simulink model "DCDC拓扑MATLAB仿真模型"  (R2024a)
settings: Solver=ode1  StartTime=0.0  StopTime=0.16  FixedStep=25e-9  MaxStep=5e-7  RelTol=1e-3
model workspace (MAT data in the model file):
  S.Coss = 1e-09
  S.Isat = 25
  S.L = 3.6e-06
  S.T_D1 = [0.71772271106 0.439813521831 0.439722845926 0.439659897498 0.439615651943 0.439584524223 0.439562966906 0.439548685103 0.439540182293 0.439536490281 0.43953700523 0.439541386891 ... (19375 elements, 25x25x31)]
  S.T_D2 = [0.717178349569 0.559937517176 0.55990263156 0.559878413607 0.55986139121 0.559849415613 0.559841122007 0.559835627482 0.559832356283 0.559830935922 0.559831134088 0.559832819881 ... (19375 elements, 25x25x31)]
  S.T_eta = [0 0 0 0 0 0 0 0 0 0 0 0 ... (19375 elements, 25x25x31)]
  S.T_fs = [30 40 75 100 125 150 200 200 200 250 250 275 ... (19375 elements, 25x25x31)]
  S.T_md = [1 1 1 1 1 1 1 1 1 1 1 1 ... (19375 elements, 25x25x31)]
  S.T_phi = [1.19741351569 0.500343703421 0.500483767979 0.500581010068 0.500649363857 0.500697454188 0.500730759931 0.500752825776 0.500765963418 0.500771668535 0.500770874014 0.500764105586 ... (19375 elements, 25x25x31)]
  S.T_pk = [1.33333333333 2.68942703114 2.73964726839 2.85027789077 2.90789704959 2.9409657645 2.48564279345 2.97524696494 3.12408185098 2.66060608601 2.77501889216 2.77086255768 ... (19375 elements, 25x25x31)]
  S.T_tr = [-1.33333333333 -2.68942703114 -2.73964726839 -2.85027789077 -2.90789704959 -2.9409657645 -2.48564279345 -2.97524696494 -3.12408185098 -2.66060608601 -2.77501889216 -2.77086255768 ... (19375 elements, 25x25x31)]
  S.bpIo = [0 0.5 1 1.5 2 2.5 3 3.5 4 4.5 5 5.5 6 6.5 7 7.5 8 8.5 9 9.5 10 10.5 11 11.5 12 12.5 13 13.5 14 14.5 15]
  S.bpVin = [24 25 26 27 28 29 30 31 32 33 34 35 36 37 38 39 40 41 42 43 44 45 46 47 48]
  S.bpVref = [24 25 26 27 28 29 30 31 32 33 34 35 36 37 38 39 40 41 42 43 44 45 46 47 48]
  S.cont1.method = 'Io-axis windowed re-solve'
  S.cont1.date = '2026-10-09'
  S.cont1.win = 'D2±0.06(扩0.15/全局), phi±5*w'
  S.cont1.skip = '等压族'
  S.dbn.policy = 'DBN4_policy'
  S.dbn.date = '2026-10-10'
  S.dbn.note = 'AI策略在线推理网格化'
  S.fsList = [30000 40000 50000 75000 100000 125000 150000 200000 250000 275000 300000]
  S.ilc.round = 1
  S.ilc.err_model = '0.054*|Vin-Vref|+0.13'
  S.ilc.lever = 'D2'
  S.ilc.date = '2026-10-09'
  S.ilc10.round = 10
  S.ilc10.basis = 'spot_def默认工况3.84A坑: 边界区D1-1q'
  S.ilc10.date = '2026-10-09'
  S.ilc11.round = 11
  S.ilc11.basis = 'spot_def阶跃平台5.74A: rows5.5/6.0 D1-1q'
  S.ilc11.date = '2026-10-09'
  S.ilc12.round = 12
  S.ilc12.basis = '真Io标定: 电阻切换负载下buck5.76A实测-3.84%'
  S.ilc12.date = '2026-10-10'
  S.ilc13.round = 13
  S.ilc13.basis = '断开后再平衡24.55(+2.28%)实测'
  S.ilc13.date = '2026-10-10'
  S.ilc2.round = 2
  S.ilc2.basis = '20点全矩阵实测'
  S.ilc2.date = '2026-10-09'
  S.ilc3.round = 3
  S.ilc3.basis = 'cal_sweep v2 17点(连续性重建表)'
  S.ilc3.date = '2026-10-09'
  S.ilc4.round = 4
  S.ilc4.basis = 'cal_sweep v3 17点残差'
  S.ilc4.date = '2026-10-09'
  S.ilc4.split = 'buck:D2x1.3; boost<2.3A:D2x1.0; boost>=2.3A:D1(死区换变量)'
  S.ilc5.round = 5
  S.ilc5.basis = 'cal_sweep v4 17点残差'
  S.ilc5.date = '2026-10-09'
  S.ilc5.detail = 'boost重载D1x2.0; buck边界4-5A加修D1; boost轻载量子踢q=25ns*fs'
  S.ilc6.round = 6
  S.ilc6.basis = 'cal_sweep v5 过冲点单量子反向'
  S.ilc6.date = '2026-10-09'
  S.ilc7.round = 7
  S.ilc7.basis = 'verify 20点终测残差'
  S.ilc7.date = '2026-10-09'
  S.ilc7.detail = 'boost row0.5 D2+2q; 对角列row0按verify误差修D2'
  S.ilc8.round = 8
  S.ilc8.basis = 'verify#2 boost轻载-5.0%过冲回调1q'
  S.ilc8.date = '2026-10-09'
  S.ilc9.round = '9c'
  S.ilc9.basis = '格点探测终选: D1净0q(+2.33%), 格距2.4V无±2%内格点'
  S.ilc9.date = '2026-10-09'
  S.td = 2e-07
  fsTab = [30 40 75 100 125 150 200 200 200 250 250 275 ... (625 elements, 25x25)]
undefined symbols (not defined in the file): DiscIntNeverNeededParam, L
libraries: spsVoltageMeasurementLib x7, spsSeriesRLCBranchLib x6, spsMosfetLib x4, spsCurrentMeasurementLib x3, spsMeanLib x2, eePowerMeasurement x2, slpidlib x1, spsDCVoltageSourceLib x1, sps_lib x1
settings Model: Creator=hp  LastModifiedBy=hp
settings DataIOCC: ReturnWorkspaceOutputs=off

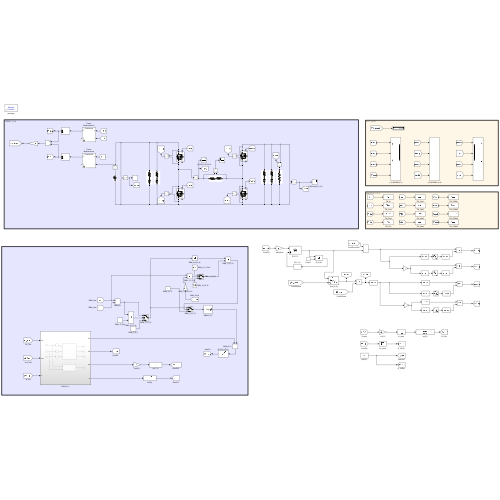
[thumbnail: Simulink's stored preview of the top-level diagram]
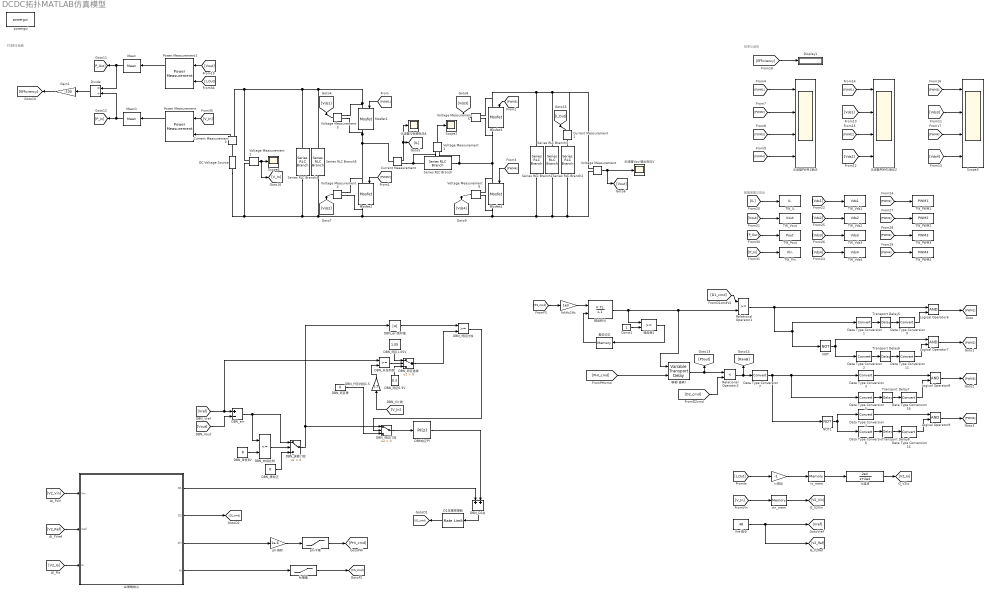
== system DCDC拓扑MATLAB仿真模型 ==
  note: FSBB主电路
  note: 效率与波形
  note: 数据收集与导出
  AI策略核心 : Subsystem
  Const1 : Constant
  Current Measurement : spsCurrentMeasurementLib/Current Measurement  PhasorSimulation=off  OutputType=Complex  PSBequivalent=0
  Current Measurement1 : spsCurrentMeasurementLib/Current Measurement  PhasorSimulation=off  OutputType=Complex  PSBequivalent=0
  Current Measurement2 : spsCurrentMeasurementLib/Current Measurement  PhasorSimulation=off  OutputType=Complex  PSBequivalent=0
  D1压摆率限制 : RateLimiter  RisingSlewLimit=50  FallingSlewLimit=-50  SampleTimeMode=inherited
  DBN_D1合 : Sum
  DBN_err : Sum  Inputs=+-
  DBN_err绝对值 : Abs  SaturateOnIntegerOverflow=off
  DBN_升压判别 : RelationalOperator  OutDataTypeStr=boolean  RndMeth=Simplest  InputSameDT=off
  DBN_升压判别1.5 : Gain  Gain=1.5
  DBN_带宽8V : Constant  Value=8
  DBN_死区0.3V : Constant  Value=0.3
  DBN_死区1.05V : Constant  Value=1.05
  DBN_死区比较 : RelationalOperator  OutDataTypeStr=boolean  RndMeth=Simplest  InputSameDT=off
  DBN_死区选择 : Switch  Criteria=u2 > Threshold  SaturateOnIntegerOverflow=off  InputSameDT=off
  DBN_死区门控 : Switch  Criteria=u2 > Threshold  SaturateOnIntegerOverflow=off  InputSameDT=off
  DBN_死区零 : Constant  Value=0
  DBN_误差门控 : Switch  Criteria=u2 > Threshold  SaturateOnIntegerOverflow=off  InputSameDT=off
  DBN_软启比较 : RelationalOperator  Operator=<=  OutDataTypeStr=boolean  RndMeth=Simplest  InputSameDT=off
  DBN_零校正 : Constant  Value=0
  DBN校正PI : slpidlib/PID Controller  Controller=PI  Form=Parallel  TimeDomain=Discrete-time  UseExternalTs=off  SampleTime=1e-5  IntegratorMethod=Forward Euler  FilterMethod=Forward Euler  ControllerParametersSource=internal  P=0.002  I=3  UseKiTs=off  D=0  UseExternalDerivativeSource=off  N=100  UseFilter=on  TunerSelectOption=Transfer Function Based (PID Tuner App)  InitialConditionSource=internal  InitialConditionForIntegrator=0  InitialConditionForFilter=0  DifferentiatorICPrevScaledInput=0  ExternalReset=none  TrackingMode=off  Kt=1  LimitOutput=on  SatLimitsSource=internal  UpperSaturationLimit=0.2  LowerSaturationLimit=-0.2  LinearizeAsGain=off  AntiWindupMode=none  Kb=1  LimitIntegrator=off  UpperIntegratorSaturationLimit=inf  LowerIntegratorSaturationLimit=-inf  POutMin=[]  POutMax=[]  IOutMin=[]  IOutMax=[]  DOutMin=[]  DOutMax=[]  NOutMin=[]  NOutMax=[]  SumOutMin=[]  SumOutMax=[]  SaturationOutMin=[]  SaturationOutMax=[]  PParamMin=[]  PParamMax=[]  IParamMin=[]  IParamMax=[]  DParamMin=[]  DParamMax=[]  NParamMin=[]  NParamMax=[]  KbParamMin=[]  KbParamMax=[]  KtParamMin=[]  KtParamMax=[]  KbOutMin=[]  KbOutMax=[]  KtOutMin=[]  KtOutMax=[]  IntegratorOutMin=[]  IntegratorOutMax=[]  FilterOutMin=[]  FilterOutMax=[]  SumI1OutMin=[]  SumI1OutMax=[]  SumI2OutMin=[]  SumI2OutMax=[]  SumI3OutMin=[]  SumI3OutMax=[]  SumI4OutMin=[]  SumI4OutMax=[]  SumDOutMin=[]  SumDOutMax=[]  DifferentiatorOutMin=[]  DifferentiatorOutMax=[]  FilterDiffOutCoefMin=[]  FilterDiffOutCoefMax=[]  ReciprocalOutMin=[]  ReciprocalOutMax=[]  SumDenOutMin=[]  SumDenOutMax=[]  SumNumOutMin=[]  SumNumOutMax=[]  DivideOutMin=[]  DivideOutMax=[]  UdiffTsProdOutMin=[]  UdiffTsProdOutMax=[]  NTsProdOutMin=[]  NTsProdOutMax=[]  UintegralTsProdOutMin=[]  UintegralTsProdOutMax=[]  UngainTsProdOutMin=[]  UngainTsProdOutMax=[]  ClampingZeroOutDataTypeStr=Inherit: Inherit via back propagation  ClampingZeroOutMin=[]  ClampingZeroOutMax=[]  FilterDenConstantOutDataTypeStr=Inherit: Inherit via back propagation  FilterDenConstantOutMin=[]  FilterDenConstantOutMax=[]  PCopyOutDataTypeStr=Inherit: Inherit via back propagation  PCopyOutMin=[]  PCopyOutMax=[]  NCopyOutDataTypeStr=Inherit: Inherit via back propagation  NCopyOutMin=[]  NCopyOutMax=[]  IntegratorContinuousStateAttributes=''  IntegratorStateMustResolveToSignalObject=off  IntegratorRTWStateStorageClass=Auto  FilterContinuousStateAttributes=''  FilterStateMustResolveToSignalObject=off  FilterRTWStateStorageClass=Auto  ParallelPVariant=InternalParameters  IdealPVariant=Disabled  IVariant=InternalParameters  DVariant=Disabled  IntegratorVariant=Discrete  SatVariant=Enabled  AWVariant=Passthrough  PCopyVariant=Disabled  TRVariant=Disabled  FdbkBlocksVariant=Forward  IdealPFdbkVariant=Disabled  SatFdbkVariant=Disabled  DerivativeFilterVariant=Disabled  NVariant=Disabled  NCopyVariant=Disabled_SignalSpec  FilterICVariant=Disabled  IntegratorICVariant=InternalICs  ExternalResetVariant=Disabled  TRSumVariant=Passthrough  SumFdbkVariant=Disabled  SumVariant=Sum_PI  TsampFilterVariant=InternalTs  TsampNgainVariant=Passthrough  TsampIntegralVariant=Disabled_SignalSpec  ExternalSaturationOutDataTypeStr=Inherit: Same as second input  DerivativeSourceVariant=Disabled
      settings: LibrarySourceBlock=simulink/Discrete/Discrete PID Controller
  DC Voltage Source : spsDCVoltageSourceLib/DC Voltage Source  Amplitude=48  Measurements=None
  Data Type Conversion{1..7,9,11,14,16} (11 alike) : DataTypeConversion  SaturateOnIntegerOverflow=off  RndMeth=Floor
  Display1 : Display
  Divide : Product  Inputs=*/
  Gain1 : Gain  Gain=-100
  Io滤波 : TransferFcn  Numerator=[2e4]  Denominator=[1 2e4]
  Logical Operator{6..9} (4 alike) : Logic  AllPortsSameDT=off  OutDataTypeStr=boolean
  Mean : spsMeanLib/Mean  Freq=50000  Vinit=0  Ts=0
  Mean1 : spsMeanLib/Mean  Freq=50000  Vinit=0  Ts=0
  Mosfet{1..4} (4 alike) : spsMosfetLib/Mosfet  Ron=4.4e-3  Lon=0  Rd=0.003  Vfd=1.5  IC=0  Rs=0.001  Cs=570e-12  Measurements=on
  NOT : Logic  Operator=NOT  IconShape=distinctive  AllPortsSameDT=off  OutDataTypeStr=boolean
  NOT1 : Logic  Operator=NOT  IconShape=distinctive  AllPortsSameDT=off  OutDataTypeStr=boolean
  Power Measurement : eePowerMeasurement/Power Measurement  LabelModeActiveChoice=Continuous  F=60  K=[0 1 2 3]  Ts=0
  Power Measurement1 : eePowerMeasurement/Power Measurement  LabelModeActiveChoice=Continuous  F=60  K=[0 1 2 3]  Ts=0
  Relational Operator1 : RelationalOperator  OutDataTypeStr=boolean  InputSameDT=off
  Relational Operator2 : RelationalOperator  Operator=<  OutDataTypeStr=boolean  InputSameDT=off
  Scope2 : Scope
  Scope3 : Scope  NumInputPorts=4
  Scope4 : Scope
  Series RLC Branch : spsSeriesRLCBranchLib/Series RLC Branch  LConnTagsString=__new0  RConnTagsString=__new0  BranchType=RL  Resistance=1.7e-3  Inductance=3.6e-6  SetiL0=off  InitialCurrent=0  Capacitance=1e-6  Setx0=off  InitialVoltage=0  Measurements=None
  Series RLC Branch1 : spsSeriesRLCBranchLib/Series RLC Branch  LConnTagsString=__new0  RConnTagsString=__new0  BranchType=RC  Resistance=2e-3  Inductance=1.5e-10  SetiL0=off  InitialCurrent=0  Capacitance=80e-6  Setx0=off  InitialVoltage=0  Measurements=Branch voltage and current
  Series RLC Branch2 : spsSeriesRLCBranchLib/Series RLC Branch  LConnTagsString=__new0  RConnTagsString=__new0  BranchType=R  Resistance=8  Inductance=L  SetiL0=off  InitialCurrent=0  Capacitance=1e-6  Setx0=off  InitialVoltage=0  Measurements=None
  Series RLC Branch3 : spsSeriesRLCBranchLib/Series RLC Branch  LConnTagsString=__new0  RConnTagsString=__new0  BranchType=RC  Resistance=0.09  Inductance=6e-9  SetiL0=off  InitialCurrent=0  Capacitance=3.667e-8  Setx0=off  InitialVoltage=0  Measurements=Branch voltage and current
  Series RLC Branch4 : spsSeriesRLCBranchLib/Series RLC Branch  LConnTagsString=__new0  RConnTagsString=__new0  BranchType=RC  Resistance=2e-3  Inductance=1.5e-10  SetiL0=off  InitialCurrent=0  Capacitance=50e-6  Setx0=off  InitialVoltage=0  Measurements=Branch voltage and current
  Series RLC Branch5 : spsSeriesRLCBranchLib/Series RLC Branch  LConnTagsString=__new0  RConnTagsString=__new0  BranchType=RC  Resistance=0.09  Inductance=6e-9  SetiL0=off  InitialCurrent=0  Capacitance=3.667e-8  Setx0=off  InitialVoltage=0  Measurements=Branch voltage and current
  TW_IL : ToWorkspace  VariableName=IL  SaveFormat=Timeseries  SampleTime=-1
  TW_PWM1 : ToWorkspace  VariableName=PWM1  SaveFormat=Timeseries  SampleTime=-1
  TW_PWM2 : ToWorkspace  VariableName=PWM2  SaveFormat=Timeseries  SampleTime=-1
  TW_PWM3 : ToWorkspace  VariableName=PWM3  SaveFormat=Timeseries  SampleTime=-1
  TW_PWM4 : ToWorkspace  VariableName=PWM4  SaveFormat=Timeseries  SampleTime=-1
  TW_Pin : ToWorkspace  VariableName=Pin  SaveFormat=Timeseries  SampleTime=-1
  TW_Pout : ToWorkspace  VariableName=Pout  SaveFormat=Timeseries  SampleTime=-1
  TW_Vds1 : ToWorkspace  VariableName=Vds1  SaveFormat=Timeseries  SampleTime=-1
  TW_Vds2 : ToWorkspace  VariableName=Vds2  SaveFormat=Timeseries  SampleTime=-1
  TW_Vds3 : ToWorkspace  VariableName=Vds3  SaveFormat=Timeseries  SampleTime=-1
  TW_Vds4 : ToWorkspace  VariableName=Vds4  SaveFormat=Timeseries  SampleTime=-1
  TW_Vout : ToWorkspace  VariableName=Vout  SaveFormat=Timeseries  SampleTime=-1
  Transport Delay{5..8} (4 alike) : TransportDelay  DelayTime=200e-9  BufferSize=500000
  Voltage Measurement{,1..6} (7 alike) : spsVoltageMeasurementLib/Voltage Measurement  PhasorSimulation=off  OutputType=Complex  PSBequivalent=0
  Vref指令 : Constant  Value=48
  fskHz2Hz : Gain  Gain=1e3
  fs限幅 : Saturate  UpperLimit=300  LowerLimit=30
  io_mem : Memory  InitialCondition=1
  io取反 : Gain  Gain=-1
  phi下限 : Saturate  UpperLimit=inf  LowerLimit=1e-7
  phi换秒 : Gain  Gain=1e-6
  powergui : sps_lib/powergui  Priority=1  SimulationMode=Discrete  SampleTime=25e-9  frequency=60  Iterations=50  frequencyindice=0  Pbase=100e6  ErrMax=1e-4  UnitsV=kV  UnitsW=MW  buscounter=0  FunctionMessages=off  echomessages=off  EnableUseOfTLC=off  CurrentSourceSwitches=off  DisableSnubberDevices=off  DisableRonSwitches=off  DisableVfSwitches=off  DisplayEquations=off  AutomaticDiscreteSolvers=off  SolverType=Tustin/Backward Euler (TBE)  Interpol=off  ExternalGateDelay=off  methode=off  Ts=100  x0status=blocks  SPID=on  SwTol=0  HookPort=off  NonlinearTolerance=1e-4  nMaxIteration=100  ContinueOnMaxIteration=off  RestoreLinks=warning  ResistiveCurrentMeasurement=off  Frange=[0:2:500]  Ylog=off  Xlog=on  ShowGrid=off  save=off  variable=ZData  structure=0  ZoomFFT=off  StartTime=0.0  cycles=1  DisplayStyle=1  fundamental=60  FreqAxis=off  MaxFrequency=1000  frequencyindicesteady=1  RmsSteady=1  display=off
  vin_mem : Memory  InitialCondition=48
  复位记忆 : Memory
  示波器IL电感电流A : Scope
  示波器PWM1驱动 : Scope  NumInputPorts=4
  示波器PWM1驱动2 : Scope  NumInputPorts=4
  示波器Vout输出电压V : Scope
  移相(查表) : VariableTransportDelay  VariableDelayType=Variable transport delay  MaximumDelay=1e-5
  锯齿满1 : RelationalOperator  OutDataTypeStr=boolean  RndMeth=Simplest  InputSameDT=off
  锯齿积分 : DiscreteIntegrator  gainval=1  ExternalReset=rising  SampleTime=25e-9  ICPrevOutput=DiscIntNeverNeededParam  ICPrevScaledInput=DiscIntNeverNeededParam
  wires:
  Voltage Measurement/1 -> [Vout], 示波器Vout输出电压V/1
  Current Measurement/1 -> [IL], 示波器IL电感电流A/1
  Voltage Measurement1/1 -> Scope2/1
  Voltage Measurement2/1 -> [V_In], Scope4/1
  [PWM2] -> Mosfet2/1
  [PWM4] -> Mosfet4/1
  [PWM3] -> Mosfet3/1
  Transport Delay5/1 -> Data Type Conversion9/1
  Data Type Conversion9/1 -> Logical Operator6/2
  Logical Operator6/1 -> [PWM1]
  Transport Delay6/1 -> Data Type Conversion11/1
  Data Type Conversion11/1 -> Logical Operator7/2
  Logical Operator7/1 -> [PWM2]
  Logical Operator9/1 -> [PWM4]
  Logical Operator8/1 -> [PWM3]
  Transport Delay7/1 -> Data Type Conversion16/1
  Transport Delay8/1 -> Data Type Conversion14/1
  Data Type Conversion16/1 -> Logical Operator8/2
  Data Type Conversion14/1 -> Logical Operator9/2
  NOT1/1 -> Data Type Conversion6/1, Data Type Conversion4/1
  Relational Operator1/1 -> Logical Operator6/1, Data Type Conversion1/1, NOT/1
  NOT/1 -> Logical Operator7/1, Data Type Conversion2/1
  Data Type Conversion3/1 -> Logical Operator8/1
  Data Type Conversion4/1 -> Logical Operator9/1
  Data Type Conversion1/1 -> Transport Delay5/1
  Data Type Conversion2/1 -> Transport Delay6/1
  Data Type Conversion5/1 -> Transport Delay7/1
  Data Type Conversion6/1 -> Transport Delay8/1
  [PWM1] -> Mosfet1/1
  Current Measurement2/1 -> Power Measurement/2
  Power Measurement1/1 -> Mean/1
  Power Measurement/1 -> Mean1/1
  Mean1/1 -> [P_In], Divide/2
  Mean/1 -> [P_Out], Divide/1
  Divide/1 -> Gain1/1
  [PWM1] -> 示波器PWM1驱动/1
  [PWM2] -> 示波器PWM1驱动/2
  [PWM3] -> 示波器PWM1驱动/3
  [PWM4] -> 示波器PWM1驱动/4
  Voltage Measurement3/1 -> [Vds1]
  Voltage Measurement4/1 -> [Vds2]
  Voltage Measurement5/1 -> [Vds3]
  [PWM1] -> 示波器PWM1驱动2/1
  [Vds1] -> 示波器PWM1驱动2/2
  [PWM2] -> 示波器PWM1驱动2/3
  [Vds2] -> 示波器PWM1驱动2/4
  [Vds4] -> Scope3/4
  [PWM4] -> Scope3/3
  [Vds3] -> Scope3/2
  [PWM3] -> Scope3/1
  Gain1/1 -> [Efficiency]
  [Efficiency] -> Display1/1
  移相(查表)/1 -> Relational Operator2/1, [PSout]
  Relational Operator2/1 -> Data Type Conversion7/1, [RawB]
  Data Type Conversion7/1 -> Data Type Conversion5/1, Data Type Conversion3/1, NOT1/1
  [D2_cmd] -> Relational Operator2/2
  [PHI_cmd] -> 移相(查表)/2
  [Vout] -> Power Measurement1/1
  [IL] -> TW_IL/1
  [Vout] -> TW_Vout/1
  [Vds1] -> TW_Vds1/1
  [Vds2] -> TW_Vds2/1
  [Vds3] -> TW_Vds3/1
  [Vds4] -> TW_Vds4/1
  [PWM1] -> TW_PWM1/1
  [PWM2] -> TW_PWM2/1
  [PWM3] -> TW_PWM3/1
  [PWM4] -> TW_PWM4/1
  [P_In] -> TW_Pin/1
  [P_Out] -> TW_Pout/1
  Current Measurement1/1 -> [I_Out]
  [I_Out] -> Power Measurement1/2
  [V_In] -> Power Measurement/1
  Voltage Measurement6/1 -> [Vds4]
  [D1_cmd] -> Relational Operator1/1
  [I_Out] -> io取反/1
  io_mem/1 -> Io滤波/1
  Io滤波/1 -> [V2_Io]
  [V_In] -> vin_mem/1
  vin_mem/1 -> [V2_Vin]
  Vref指令/1 -> [Vref], [V2_Ref]
  fs限幅/1 -> [FS_cmd]
  phi换秒/1 -> phi下限/1
  phi下限/1 -> [PHI_cmd]
  [FS_cmd] -> fskHz2Hz/1
  fskHz2Hz/1 -> 锯齿积分/1
  锯齿积分/1 -> 锯齿满1/1, 移相(查表)/1, Relational Operator1/2
  Const1/1 -> 锯齿满1/2
  锯齿满1/1 -> 复位记忆/1
  复位记忆/1 -> 锯齿积分/2
  io取反/1 -> io_mem/1
  [Vref] -> DBN_升压判别/1, DBN_err/1
  [Vout] -> DBN_err/2
  AI策略核心/1(D1) -> DBN_D1合/1
  AI策略核心/2(D2) -> [D2_cmd]
  AI策略核心/3(phi) -> phi换秒/1
  AI策略核心/4(fs) -> fs限幅/1
  [V2_Vin] -> AI策略核心/1(Vin)
  [V2_Ref] -> AI策略核心/2(Vref)
  [V2_Io] -> AI策略核心/3(Io)
  DBN_软启比较/1 -> DBN_误差门控/2
  DBN_零校正/1 -> DBN_误差门控/3
  DBN_D1合/1 -> D1压摆率限制/1
  D1压摆率限制/1 -> [D1_cmd]
  DBN_err/1 -> DBN_误差门控/1, DBN_软启比较/1
  DBN_带宽8V/1 -> DBN_软启比较/2
  DBN校正PI/1 -> DBN_D1合/2
  DBN_误差门控/1 -> DBN_err绝对值/1, DBN_死区门控/1
  DBN_死区零/1 -> DBN_死区门控/3
  DBN_死区门控/1 -> DBN校正PI/1
  [V_In] -> DBN_升压判别1.5/1
  DBN_升压判别1.5/1 -> DBN_升压判别/2
  DBN_死区1.05V/1 -> DBN_死区选择/1
  DBN_死区0.3V/1 -> DBN_死区选择/3
  DBN_升压判别/1 -> DBN_死区选择/2
  DBN_死区选择/1 -> DBN_死区比较/2
  DBN_err绝对值/1 -> DBN_死区比较/1
  DBN_死区比较/1 -> DBN_死区门控/2
  connections:
  Series RLC Branch2/RConn1 -- Voltage Measurement/LConn2 -- Series RLC Branch3/RConn1 -- Voltage Measurement6/LConn2 -- Mosfet4/RConn1 -- Voltage Measurement4/LConn2 -- Mosfet2/RConn1 -- Series RLC Branch5/RConn1 -- Series RLC Branch4/RConn1 -- Voltage Measurement2/LConn2 -- DC Voltage Source/LConn1 -- Series RLC Branch1/RConn1
  Series RLC Branch3/LConn1 -- Current Measurement1/RConn1 -- Voltage Measurement/LConn1 -- Voltage Measurement5/LConn1 -- Mosfet3/LConn1 -- Series RLC Branch1/LConn1
  Series RLC Branch/RConn1 -- Voltage Measurement6/LConn1 -- Mosfet4/LConn1 -- Voltage Measurement5/LConn2 -- Mosfet3/RConn1 -- Voltage Measurement1/LConn2
  Current Measurement/RConn1 -- Voltage Measurement1/LConn1 -- Series RLC Branch/LConn1
  Mosfet1/RConn1 -- Voltage Measurement3/LConn2 -- Voltage Measurement4/LConn1 -- Mosfet2/LConn1 -- Current Measurement/LConn1
  Voltage Measurement2/LConn1 -- Current Measurement2/RConn1 -- Series RLC Branch4/LConn1 -- Series RLC Branch5/LConn1 -- Voltage Measurement3/LConn1 -- Mosfet1/LConn1
  DC Voltage Source/RConn1 -- Current Measurement2/LConn1
  Current Measurement1/LConn1 -- Series RLC Branch2/LConn1

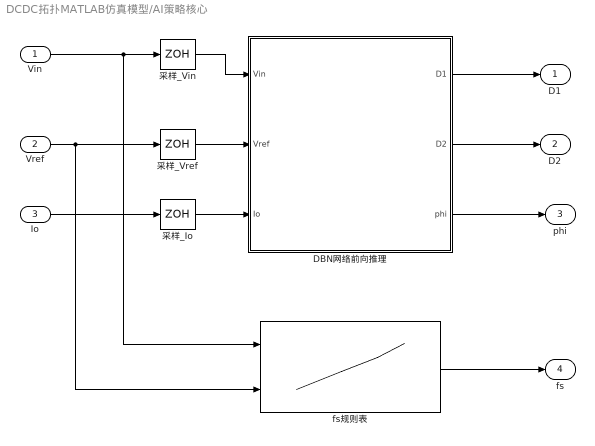
== system DCDC拓扑MATLAB仿真模型/AI策略核心 ==
  Vin : Inport
  Vref : Inport  Port=2
  Io : Inport  Port=3
  DBN网络前向推理 : MATLAB Function  TreatAsAtomicUnit=on
  fs规则表 : Lookup_n-D  BreakpointsForDimension1=S.bpVin  BreakpointsForDimension2=S.bpVref  BreakpointsForDimension3=[5, 7]  Table=fsTab  ExtrapMethod=Clip  InternalRulePriority=Speed  RndMeth=Simplest
      settings: InputPortMap=u0,u1
  采样_Io : ZeroOrderHold  SampleTime=1e-5
  采样_Vin : ZeroOrderHold  SampleTime=1e-5
  采样_Vref : ZeroOrderHold  SampleTime=1e-5
  D1 : Outport
  D2 : Outport  Port=2
  phi : Outport  Port=3
  fs : Outport  Port=4
  wires:
  采样_Vin/1 -> DBN网络前向推理/1(Vin)
  采样_Vref/1 -> DBN网络前向推理/2(Vref)
  采样_Io/1 -> DBN网络前向推理/3(Io)
  DBN网络前向推理/1(D1) -> D1/1
  DBN网络前向推理/2(D2) -> D2/1
  DBN网络前向推理/3(phi) -> phi/1
  fs规则表/1 -> fs/1
  Vin/1 -> 采样_Vin/1, fs规则表/1
  Vref/1 -> fs规则表/2, 采样_Vref/1
  Io/1 -> 采样_Io/1

== matlab function DCDC拓扑MATLAB仿真模型/AI策略核心/DBN网络前向推理 ==
  data: Vin input; D1 output; Vref input; Io input; D2 output; phi output
function [D1, D2, phi] = dbn_policy(Vin, Vref, Io)
%#codegen
% DBN策略网络 · 真在线前向推理 (DBN6直接监督训练(Xavier+Adam,RBM饱和实证后弃预训练) 2026-10-10, 脚本fsbb_dbn5.m)
% 架构: [Vin,Vref,Io,Vref/Vin] -> 16 sigmoid -> 16 sigmoid -> 3 线性
% 训练: CD-1预训练+加权岭回归+加权BP; 标签=LUT4V(r11)约束最优表, Io<=8域
%   加权: buck轻载x6/等压x3/boost轻载x3 (治buck轻载D1偏粗+等压φ斜坡欠拟合)
% 三分区: B=buck(Vin>Vref+0.5) / E=等压带 / O=boost
% 输出: D1,D2=桥臂占空比, phi=移相(µs); fs为列恒定规则量, 由fs规则表块给出
% 包络保护: 输入投影进训练域, boost按300W包络限Io, 输出投影可行盒 -> 永无NaN

% ---------- netB buck分区 ----------
W1_B = [0.09560433 -0.2102087 -1.092915 -8.136814 -0.6577125 20.22259 -1.055329 0.9708207 3.19219 -0.4056949 1.426285 9.849862 6.506143 -5.503647 1.152061 4.680168;-0.1972165 0.1524808 1.48993 7.646841 1.271195 -10.40615 1.617461 -1.142764 -3.043919 0.6013724 -0.8584289 -7.485821 -8.606891 6.117011 -2.870498 -4.635286;-8.835936 -4.903688 3.196881 -5.868281 -2.040477 6.651628 -0.58446 -9.067274 -2.356474 3.523997 -2.81016 -0.9004363 -0.6001857 -3.564277 -0.8138937 -1.471235;0.1517554 -0.232312 -4.104722 2.285444 -1.88291 3.746562 -0.3180625 1.151273 -1.72326 -1.194088 -0.7909105 -6.307744 14.1946 -2.701206 -1.403806 1.403795];
b1_B = [-5.792 -8.747525 2.57083 12.50179 -3.238703 -21.29814 0.2327088 -8.814916 6.129884 3.291437 0.0009636891 12.53324 -5.078174 -4.002129 -0.6885032 -4.234402];
W2_B = [-0.6424536 -0.980142 -3.47526 -0.8581849 -4.302394 0.06394036 -1.797014 -5.298015 -0.7433495 1.325448 0.5203817 3.485016 0.741289 -3.414191 -0.8669285 -11.29654;3.222887 11.87229 -2.182464 -0.3629083 4.256677 -0.1623975 2.571575 -7.616158 -3.572853 0.02864427 3.089713 -7.015255 -5.368082 -4.810077 -1.022758 9.94359;1.357645 2.861197 -1.083953 5.005029 1.916258 2.222117 -2.988828 -1.042833 -0.3763012 -5.206152 0.0524359 -3.221319 4.74484 -0.1031338 1.640056 7.260228;0.4078975 -0.637527 0.5764574 -0.4057369 0.2550449 -0.1793036 -0.2856404 9.925458 0.8256588 0.8696184 0.05082674 0.3120586 -0.2215763 0.5356647 0.3215325 -0.2788634;2.504541 0.01980779 0.9669968 0.8989408 -2.741065 -1.117742 -9.292027 -3.471328 -0.9749411 2.265912 0.3073803 3.135268 -1.46336 -4.754087 -0.7719506 -5.539488;-0.3538728 0.6410382 -0.8867305 1.901654 -0.8844021 -0.04394435 0.9346432 1.653624 -1.824912 -1.091243 -0.1856008 0.392988 -0.06171568 -19.91326 0.2573506 0.1947155;-2.360375 1.161235 0.9783518 -2.098556 -2.430294 -0.9162419 -1.04287 -0.6944866 1.403863 -4.597777 -2.140697 0.8911189 0.9230895 4.253032 -0.6212465 -3.773626;-2.926501 -3.073559 -3.134998 -0.5231291 2.624952 2.449437 -0.752771 -0.5726463 -0.9599995 -0.2173539 0.9941455 5.644538 -3.672302 -5.288638 -0.4493547 29.48987;0.8063296 -3.771385 1.419403 0.3905247 -0.04960936 -0.2972454 0.9106917 0.6662481 -1.499891 0.9546305 1.069848 -2.500684 -7.354378 2.680403 0.4593508 1.90041;-1.997795 6.040323 -0.05892463 -1.685093 5.177251 2.108692 0.6808559 11.37892 -0.03726176 0.1818881 0.08614405 -2.927698 5.921836 20.56637 -1.078405 -5.426179;1.975887 -0.2092842 -0.3036289 0.26076 -2.868536 -0.8277971 -0.02798549 1.238514 -0.2912258 -1.972965 0.4477454 0.7854728 -2.859331 0.5924792 -2.192759 7.868733;0.1811819 -2.838926 0.9656826 -0.6815445 3.049429 -0.8457803 0.05419922 0.05275373 -0.5001539 0.9430978 0.151192 0.9267854 -4.931051 -0.07650615 0.2134373 -1.498354;0.7780109 -6.885549 2.895925 2.774903 3.41664 -1.411374 -0.3157284 -0.7148287 1.35457 2.125169 0.5777939 0.9602231 -11.5242 -0.2951642 3.249785 -1.198246;-1.281158 -2.771266 1.376839 3.099394 0.1175263 -0.2095641 1.225214 -2.607991 -2.233689 -3.775781 -0.4512342 -1.817599 -2.494865 1.01748 1.115422 4.150498;1.624013 0.9811241 1.675182 -4.855052 1.181495 0.0360339 -2.315075 0.7141644 4.397918 0.08957265 0.3406312 0.5658766 0.08565086 1.193919 -1.229547 0.4617241;-3.574682 -2.930259 0.4348486 5.214306 -0.1799769 -1.878402 -1.653529 -5.118598 -5.332303 -1.583739 -0.6728597 0.42586 -1.68062 -2.571596 -1.830005 -1.860416];
b2_B = [0.3991152 1.654256 0.4694036 -0.08192317 0.5210717 0.09345862 1.294651 0.3875052 -0.2405838 0.1764202 -1.807871 -3.835826 6.470826 3.051092 -0.5157873 -1.224625];
Wo_B = [-0.1579496 -3.463938 -0.4431134;-2.784236 -6.699247 -2.027433;-0.5839332 -0.8702263 2.19358;-0.7741133 -2.429405 0.6784985;1.362505 3.554812 -1.063732;-0.09578426 2.123025 3.857045;-0.6125204 -3.304689 1.426018;0.6097742 3.004456 1.7265;-0.293974 -2.215623 0.6828922;0.4778928 -1.52144 7.828323;-3.608602 -0.3549101 -0.873984;-0.3389829 -3.348472 0.09988118;2.49378 4.432909 -2.171237;-0.6451911 -2.847513 -1.621644;1.466551 3.72232 -1.578729;0.1626644 2.188757 -0.07472723];
c0_B= [0.9838465 0.5788606 -1.040367];
mx_B= [40.26529 31.72164 7.652247 0.794269];
sx_B= [5.767407 5.77382 4.276733 0.1243147];
my_B= [0.553016 0.6076111 0.4152078];
sy_B= [0.1408473 0.07821521 0.4352623];
% ---------- netE 等压带分区 ----------
W1_E = [0.8687102 6.488779 -4.202644 6.103957 0.2959282 8.556436 3.181142 0.4918098 -2.371691 -5.539834 0.8260288 -0.03310489 -3.853129 0.5736928 -4.894305 1.624501;0.76802 6.406573 -4.16915 6.248227 0.9532152 8.349091 3.466705 0.6868531 -2.782769 -5.827239 0.3614963 -0.2052322 -3.357931 0.5507997 -5.164385 1.78793;-0.4156608 6.402252 0.7639 -14.06762 7.517165 0.9946808 4.374741 3.378211 -4.016703 -5.827972 -40.21262 -1.715275 7.250412 -20.29872 4.488919 11.35394;-0.02716803 0.2599169 0.1382474 -0.3706387 -0.04810627 0.1126234 0.3050103 0.1529413 0.1835715 0.09058718 -0.4277605 -0.6771861 0.02480904 -0.5395588 -0.5966558 -0.2021638];
b1_E = [1.214867 8.5566 11.11962 -10.51447 8.567084 -18.83812 13.51992 5.817085 -7.636217 -18.01716 0.9523958 -1.004894 8.603222 -0.6490367 9.521392 16.24572];
W2_E = [-7.477788 4.377367 -5.066105 2.087515 -2.850699 1.603155 -0.9145926 3.517907 1.887275 -1.218283 2.66135 1.294502 -1.555509 -1.434131 -3.944127 2.952636;1.572412 -0.9596428 4.490992 0.1349776 1.178356 -4.271457 0.2371773 -2.256694 -0.1465256 2.131451 -1.23484 -3.580222 -0.9741769 -0.1925778 -0.09876817 0.6024158;5.364982 -1.634812 0.9540648 -5.947429 -5.232487 -0.4317926 -0.7864889 2.850873 0.8618857 -5.41347 0.2075044 1.892952 1.37698 1.100661 1.378364 -1.246826;-14.56837 -5.203606 -4.92141 2.937767 -4.421117 -18.97969 -0.7803484 4.964627 0.2776394 7.007463 -3.286702 3.563002 0.307172 0.8949501 0.5438612 6.333067;2.758612 -0.1184936 20.80365 -2.352003 7.823181 6.916454 1.038201 -2.824526 -0.6868771 2.599624 3.055313 -4.745298 2.844676 -2.122928 -2.203252 -3.982051;5.212056 3.340105 -3.44923 -3.252466 4.342586 2.669515 0.2536292 -8.418508 -0.6132951 1.44053 -13.52705 -7.399386 -0.9670425 -0.2476921 -51.52762 -4.974516;16.45976 3.183323 -0.06614504 -1.194062 -1.645007 0.4564601 0.4933043 -3.094398 0.04234828 0.1920126 1.484252 0.7849407 -1.470945 -0.9939989 1.867266 2.874936;3.766005 0.7450877 7.312702 -2.25361 2.572309 5.35478 1.384966 -0.4067083 -1.97966 3.271455 3.477393 -0.4028278 1.721037 2.414378 -2.48097 -1.761718;-6.797488 -2.828444 -6.749211 -74.24461 3.8022 -5.05077 -1.005018 4.597084 0.573895 -0.5484883 -0.8201514 -5.686085 7.824509 1.108694 -0.4115317 6.413057;-12.58369 1.899071 -4.924054 -7.066773 15.89929 11.65909 0.2717794 10.5077 -0.1378848 -10.21189 -4.243067 2.689568 -4.591162 -0.3377537 2.099463 6.715869;-2.805605 -5.309648 -1.36248 2.110392 -2.697435 2.281813 0.6043971 1.065571 3.236208 -12.47747 -0.906607 1.443956 0.3755221 -0.6815628 0.62765 1.001954;-3.117107 2.469092 -3.766047 1.428185 -4.184276 0.6709935 -2.421416 0.9600136 1.679417 -10.59903 -2.919156 1.420394 -5.261986 -3.21212 -1.579926 -1.15894;12.35711 3.347967 12.02989 -9.535385 -0.6113785 -1.54432 0.7310258 -25.12855 -1.677896 4.361344 3.215806 -10.81934 0.5857394 -1.088445 0.3897201 -4.844976;-1.523959 -4.840789 -0.7048018 1.629605 -0.9637606 1.303731 1.514646 0.7344346 1.759397 -5.314079 0.6998129 1.62602 0.2069579 2.218481 -0.6294821 -1.024262;4.216716 -3.561885 8.063233 -16.78168 17.72526 -1.991655 -0.03614734 -5.197618 -0.08721939 10.40447 -0.1785647 -5.308615 -0.7593139 0.4845765 1.545269 -5.065281;5.025169 1.345727 18.63976 -1.719338 5.916613 6.596827 0.1490323 -2.726667 -2.194988 0.6611103 9.410709 -3.210261 2.421886 -0.5750368 -2.84058 -3.404421];
b2_E = [-0.04295921 0.4279668 -0.06099872 0.08077504 -1.685141 2.451188 0.07488259 -0.9833854 -0.5519185 -1.758439 -0.01171036 1.297805 -0.5179021 0.4234589 0.1212619 -0.4754727];
Wo_E = [4.602225 4.653459 -0.3179917;-1.886251 -1.938442 -0.7205369;3.541915 3.569343 -0.00486989;-4.417653 -4.455436 -0.1205642;-3.079122 -3.123956 0.2314251;-1.775017 -1.780002 0.1637457;1.350867 1.286338 3.621825;-3.929178 -3.967025 0.2097626;-0.4284529 -0.4130562 -4.663121;1.700101 1.704669 -4.160785;-6.151353 -6.193929 0.2727013;6.2043 6.275661 -0.3733803;2.615724 2.649705 0.1720188;-1.899409 -1.983652 3.476383;5.629233 5.704506 -0.1267678;-4.881965 -4.972495 0.3967534];
c0_E= [0.01279763 0.09558599 -0.02288011];
mx_E= [36 36 7.75 1];
sx_E= [7.215915 7.215915 4.330609 1];
my_E= [0.7591244 0.7577011 1.014533];
sy_E= [0.05344711 0.05327648 0.5544234];
% ---------- netO boost分区 ----------
W1_O = [1.166687 1.634208 -26.25007 -2.196641 -3.707355 -2.899093 -0.6890143 -3.534197 -1.558456 1.61548 -8.084228 8.598365 0.8475441 3.412596 -0.9529444 -6.102449;-0.9275863 -1.463943 28.09734 2.932965 1.690365 2.727954 1.575852 2.759548 0.9553501 -1.905148 6.714971 -5.829413 -0.5716528 -2.543549 0.07598382 6.618692;3.53107 -0.6517366 -0.9499759 -0.519107 0.1555406 3.58535 -0.4703955 5.14823 -3.313984 7.413182 -7.167878 -3.36604 0.1285425 -0.1908854 1.374792 -2.595477;0.3093429 -1.016448 -4.688949 -0.9238681 4.974052 -0.8880755 -2.384261 -1.492858 -1.488719 1.4723 -5.798669 3.478437 -2.011764 -4.084038 -0.2223285 -4.392692];
b1_O = [4.146893 -3.716447 12.1455 -2.144462 4.686571 3.635428 0.3915236 2.885802 2.044519 7.203908 -3.51686 0.6749363 0.7655944 -4.05796 1.779268 -0.826674];
W2_O = [-0.543638 0.9874986 1.616888 2.484575 1.051016 -1.685497 9.917357 0.7204378 0.5941047 -0.5427948 4.303518 -13.97797 -0.07824607 -3.585724 -2.158289 -1.298964;-1.509273 2.653036 -6.003145 1.943032 9.801548 0.4904396 -4.24235 1.193472 2.027044 -0.5678418 -1.799253 9.436654 2.595209 4.194414 1.471981 -2.601804;0.5743247 -1.076129 -0.4280598 2.480167 1.897141 0.05959839 -0.1906791 3.960238 4.548856 -0.2511781 -0.07511974 -0.04896922 0.7984599 0.2128039 -0.2292677 -0.692862;1.475593 2.262783 -2.279659 2.640311 -6.755687 -1.14405 -1.096117 -0.5122592 -2.642773 1.285729 1.385406 -1.330968 -4.287627 1.361448 0.6689465 0.1610987;1.852798 1.094231 -0.5072462 -5.190397 -6.425553 0.3275779 -0.1520584 -3.133257 -6.379865 0.02021026 0.3587008 0.3012059 -1.047772 -0.3786371 0.04910487 1.736028;-1.615897 -0.206169 5.500525 -0.9260817 4.145941 0.8330136 5.129912 0.9840496 4.528981 -1.367898 2.401426 -4.10303 0.7230709 -0.2147545 0.1333534 -0.9479471;-0.5984088 -6.20108 -2.364607 2.949457 7.428369 0.470871 0.9005439 1.377754 1.746585 -0.4876313 -2.702698 -2.040967 0.1629725 -0.1187561 -0.9059062 -1.97866;-0.5698668 -0.8234448 1.237497 1.191379 -2.104863 0.1774358 -8.382301 3.719465 4.362246 -1.826511 -2.062484 -9.21146 1.746382 -7.605194 -4.80337 -2.299133;-0.1553445 -0.1203695 -3.093007 -6.551404 -2.138018 -0.2147934 -0.8319643 -1.963785 -5.258413 0.2255649 -1.601769 3.110451 0.02865037 1.291929 0.9079693 0.8167385;3.235331 0.5979005 -6.081422 5.689245 2.395988 0.6134156 23.04943 4.811944 2.901781 2.642427 2.894843 -10.24435 0.5405547 0.2169209 -2.382885 -1.455031;-0.3385413 -0.4598451 -1.1014 0.2867788 0.08435256 -0.3407239 -2.526461 0.9172145 3.739571 -0.1098131 -3.155885 9.403064 -0.3409335 0.3562731 -1.083251 -0.909064;0.1144054 0.9983101 5.106238 -3.175789 -0.7924275 0.1172985 -1.257779 -3.303221 -3.01285 1.159691 0.536155 0.05553541 -1.342709 -0.8286728 1.231603 0.9758357;-2.786969 -1.91014 5.21125 -0.07825397 -6.252928 0.93636 0.6847653 -1.527477 0.2562477 0.5653937 1.522381 -0.1699287 -1.425742 -0.03033537 0.553366 1.014837;-12.55089 4.043606 0.3017281 -9.343027 -13.47037 0.7756375 0.839089 -6.029277 -11.18965 -2.084893 1.672203 -1.368507 -1.672516 -0.3576598 0.7533413 7.199143;-0.4283863 -0.003401899 2.623277 6.086506 4.221306 -0.08931896 0.883116 4.438592 2.244463 -0.02655831 -0.8881515 -1.320569 1.104852 -0.055539 -0.9422878 -0.9289631;0.07391611 -0.8791575 -0.005258738 0.9337907 5.549889 -0.1746889 0.05817595 -2.38703 -4.199413 1.241252 1.195613 0.484081 -0.6499711 1.598894 -0.3570141 -4.308544];
b2_O = [-1.291696 -2.514526 0.9971383 0.421179 1.48215 -0.0762833 1.269049 -2.121707 1.844378 0.4086856 -0.9169433 0.9746297 -0.8338121 -0.6762498 0.8428862 1.623319];
Wo_O = [-0.782854 -1.806263 2.217243;-0.5075165 -4.605253 5.219332;2.15659 2.139982 0.524831;-1.411994 -2.358743 -0.1109297;0.1767176 0.4806217 -1.297739;-2.615528 -1.774808 1.628059;1.032635 0.9836415 1.360333;-0.3577451 -1.282877 4.012986;1.507922 2.891006 -6.67688;-0.5306917 -2.672349 -0.7599057;0.9790112 2.534584 -0.2108256;-0.6153128 1.959283 0.1452227;-0.1330224 -1.871284 -0.5275731;0.1819581 -3.098258 -2.610988;-3.029714 0.5322406 -0.3771162;0.2662966 -0.3895114 -1.923294];
c0_O= [-1.167329 -0.6800091 0.7834842];
mx_O= [32.20606 39.90215 6.961883 1.259833];
sx_O= [5.842601 5.867935 4.051607 0.2057379];
my_O= [0.8434158 0.5255383 1.030493];
sy_O= [0.1354036 0.0905518 0.3858575];
xV = min(max(Vin ,23.5),48.5);      % 输入投影到训练域(Io域已收到8)
xR = min(max(Vref,23.5),48.5);
xI = min(max(Io  ,0),8);
if xR > xV + 0.5                    % boost族300W包络
    xI = min(xI, 300/xR);
end
if Vin > Vref + 0.5                 % 分区路由(与训练一致)
    y = fwd(xV, xR, xI, W1_B,b1_B,W2_B,b2_B,Wo_B,c0_B,mx_B,sx_B,my_B,sy_B);
elseif Vin < Vref - 0.5
    y = fwd(xV, xR, xI, W1_O,b1_O,W2_O,b2_O,Wo_O,c0_O,mx_O,sx_O,my_O,sy_O);
else
    y = fwd(xV, xR, xI, W1_E,b1_E,W2_E,b2_E,Wo_E,c0_E,mx_E,sx_E,my_E,sy_E);
end
D1  = min(max(y(1),0.02),0.95);     % 可行盒投影
D2  = min(max(y(2),0.05),0.90);
phi = min(max(y(3),0.1),3);

function y = fwd(Vin, Vref, Io, W1,b1,W2,b2,Wo,c0,mx,sx,my,sy)
x  = [Vin, Vref, Io, Vref/Vin];
xn = (x - mx)./sx;                  % 输入标准化(训练统计量)
a1 = 1./(1+exp(-(xn*W1 + b1)));     % 隐层1 sigmoid
a2 = 1./(1+exp(-(a1*W2 + b2)));     % 隐层2 sigmoid
y  = (a2*Wo + c0).*sy + my;         % 线性读出+反标准化
